simulink model "simulation"  (R2016b)
settings: Solver=VariableStepAuto  StartTime=0.0  StopTime=10.0  RelTol=1e-3
libraries: simulink x4
settings Model: Creator=Hosein  LastModifiedBy=Hosein

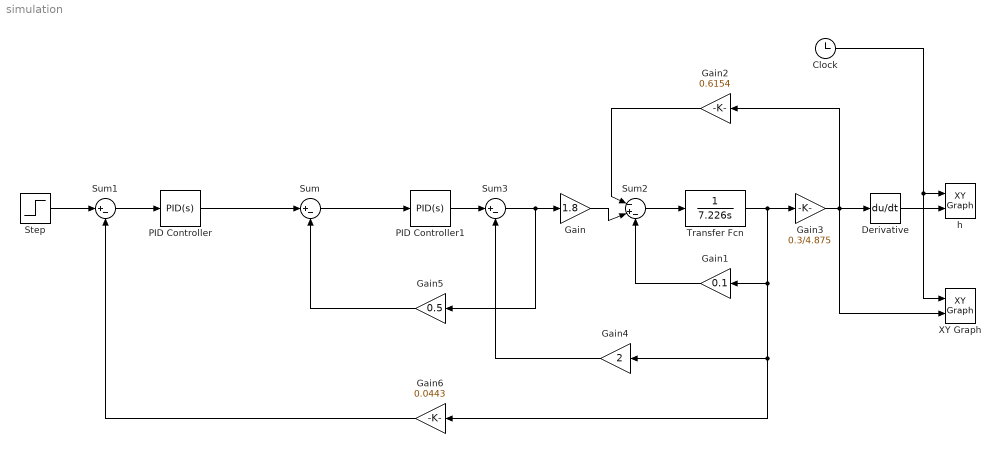
== system simulation ==
  Clock : Clock
  Derivative : Derivative
  Gain : Gain  Gain=1.8
  Gain1 : Gain  Gain=0.1
  Gain2 : Gain  Gain=0.6154
  Gain3 : Gain  Gain=0.3/4.875
  Gain4 : Gain  Gain=2
  Gain5 : Gain  Gain=0.5
  Gain6 : Gain  Gain=0.0443
  PID Controller : simulink/Continuous/PID Controller  Controller=PID  TimeDomain=Continuous-time  SampleTime=-1  IntegratorMethod=Forward Euler  FilterMethod=Forward Euler  Form=Parallel  UseFilter=on  ControllerParametersSource=internal  P=100  I=40  D=0  N=100  InitialConditionSource=internal  InitialConditionForIntegrator=0  InitialConditionForFilter=0  ExternalReset=none  LimitOutput=off  UpperSaturationLimit=inf  LowerSaturationLimit=-inf  LinearizeAsGain=on  AntiWindupMode=none  Kb=1  TrackingMode=off  Kt=1  PParamMin=[]  PParamMax=[]  IParamMin=[]  IParamMax=[]  DParamMin=[]  DParamMax=[]  NParamMin=[]  NParamMax=[]  KbParamMin=[]  KbParamMax=[]  KtParamMin=[]  KtParamMax=[]  POutMin=[]  POutMax=[]  IOutMin=[]  IOutMax=[]  DOutMin=[]  DOutMax=[]  NOutMin=[]  NOutMax=[]  KbOutMin=[]  KbOutMax=[]  KtOutMin=[]  KtOutMax=[]  IntegratorOutMin=[]  IntegratorOutMax=[]  FilterOutMin=[]  FilterOutMax=[]  SumOutMin=[]  SumOutMax=[]  SumI1OutMin=[]  SumI1OutMax=[]  SumI2OutMin=[]  SumI2OutMax=[]  SumI3OutMin=[]  SumI3OutMax=[]  SumDOutMin=[]  SumDOutMax=[]  SaturationOutMin=[]  SaturationOutMax=[]  IntegratorContinuousStateAttributes=''  IntegratorStateMustResolveToSignalObject=off  IntegratorRTWStateStorageClass=Auto  FilterContinuousStateAttributes=''  FilterStateMustResolveToSignalObject=off  FilterRTWStateStorageClass=Auto  DifferentiatorICPrevScaledInput=0  DifferentiatorOutMin=[]  DifferentiatorOutMax=[]
  PID Controller1 : simulink/Continuous/PID Controller  Controller=PID  TimeDomain=Continuous-time  SampleTime=-1  IntegratorMethod=Forward Euler  FilterMethod=Forward Euler  Form=Parallel  UseFilter=on  ControllerParametersSource=internal  P=10  I=6  D=0  N=100  InitialConditionSource=internal  InitialConditionForIntegrator=0  InitialConditionForFilter=0  ExternalReset=none  LimitOutput=off  UpperSaturationLimit=inf  LowerSaturationLimit=-inf  LinearizeAsGain=on  AntiWindupMode=none  Kb=1  TrackingMode=off  Kt=1  PParamMin=[]  PParamMax=[]  IParamMin=[]  IParamMax=[]  DParamMin=[]  DParamMax=[]  NParamMin=[]  NParamMax=[]  KbParamMin=[]  KbParamMax=[]  KtParamMin=[]  KtParamMax=[]  POutMin=[]  POutMax=[]  IOutMin=[]  IOutMax=[]  DOutMin=[]  DOutMax=[]  NOutMin=[]  NOutMax=[]  KbOutMin=[]  KbOutMax=[]  KtOutMin=[]  KtOutMax=[]  IntegratorOutMin=[]  IntegratorOutMax=[]  FilterOutMin=[]  FilterOutMax=[]  SumOutMin=[]  SumOutMax=[]  SumI1OutMin=[]  SumI1OutMax=[]  SumI2OutMin=[]  SumI2OutMax=[]  SumI3OutMin=[]  SumI3OutMax=[]  SumDOutMin=[]  SumDOutMax=[]  SaturationOutMin=[]  SaturationOutMax=[]  IntegratorContinuousStateAttributes=''  IntegratorStateMustResolveToSignalObject=off  IntegratorRTWStateStorageClass=Auto  FilterContinuousStateAttributes=''  FilterStateMustResolveToSignalObject=off  FilterRTWStateStorageClass=Auto  DifferentiatorICPrevScaledInput=0  DifferentiatorOutMin=[]  DifferentiatorOutMax=[]
  Step : Step  Time=0  After=4  SampleTime=0
  Sum : Sum  Inputs=|+-
  Sum1 : Sum  Inputs=|+-
  Sum2 : Sum  Inputs=|-+-
  Sum3 : Sum  Inputs=|+-
  Transfer Fcn : TransferFcn  Denominator=[7.226 0]
  XY Graph : simulink/Sinks/XY Graph  xmin=0  xmax=8  ymin=0  ymax=10  st=0
  "h " : simulink/Sinks/XY Graph  xmin=0  xmax=12  ymin=-1  ymax=12  st=-1
  wires:
  PID Controller/1 -> Sum/1
  Sum/1 -> PID Controller1/1
  Step/1 -> Sum1/1
  Sum1/1 -> PID Controller/1
  Gain5/1 -> Sum/2
  PID Controller1/1 -> Sum3/1
  Sum3/1 -> Gain5/1, Gain/1
  Transfer Fcn/1 -> Gain6/1, Gain4/1, Gain1/1, Gain3/1
  Gain3/1 -> XY Graph/2, Derivative/1, Gain2/1
  Gain/1 -> Sum2/2
  Gain2/1 -> Sum2/1
  Gain1/1 -> Sum2/3
  Sum2/1 -> Transfer Fcn/1
  Gain4/1 -> Sum3/2
  Gain6/1 -> Sum1/2
  Derivative/1 -> "h "/2
  Clock/1 -> XY Graph/1, "h "/1
